simulink model "power_theft_simulink_2"  (R2026a)
settings: Solver=ode23t  StopTime=6  MaxStep=1e-4
libraries: fl_lib x14, nesl_utility x7, ee_lib x1
settings Model: Creator=LAKSHMAN  LastModifiedBy=LAKSHMAN

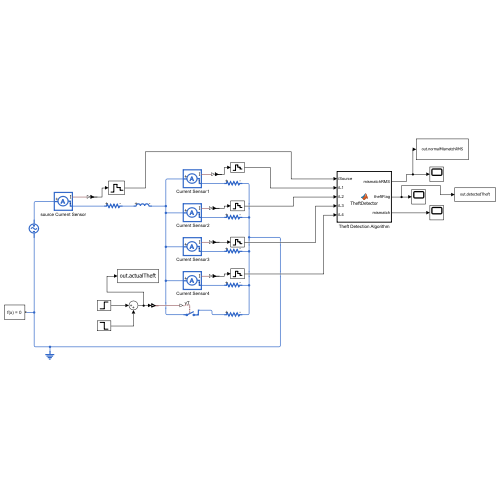
[thumbnail: Simulink's stored preview of the top-level diagram]
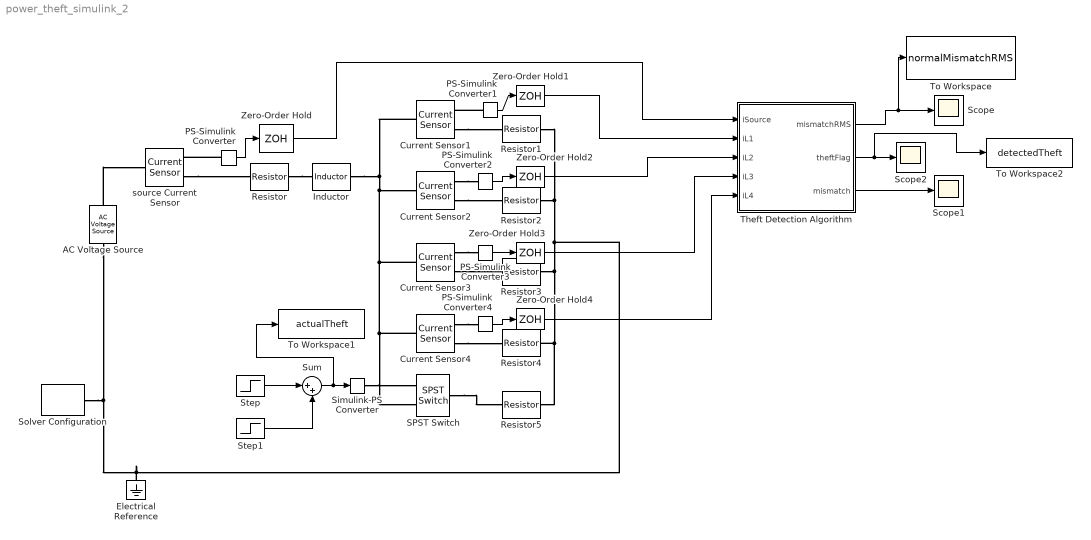
== system power_theft_simulink_2 ==
   Current Sensor{1..4} (4 alike) : fl_lib/Electrical/Electrical Sensors/Current Sensor
  AC Voltage Source : fl_lib/Electrical/Electrical Sources/AC Voltage Source  amp=325.27 V  shift=0 deg  frequency=50 Hz
  Electrical Reference : fl_lib/Electrical/Electrical Elements/Electrical Reference
  Inductor : fl_lib/Electrical/Electrical Elements/Inductor  l=1e-6 H  r=0 Ohm  g=1e-9 1/Ohm  i_specify=off  i_priority=None  i=0 A  i_nominal_specify=off  i_nominal_value=1  i_nominal_unit=A  v_specify=off  v_priority=None  v=0 V  v_nominal_specify=off  v_nominal_value=1  v_nominal_unit=V  i_L_specify=off  i_L_priority=High  i_L=0 A  i_L_nominal_specify=off  i_L_nominal_value=1  i_L_nominal_unit=A
  PS-Simulink Converter{,1..4} (5 alike) : nesl_utility/PS-Simulink Converter  PhysicalDomain=network_engine_domain  SubClassName=ps_output  LeftPortType=input  RightPortType=output  PseudoPeriodic=off  Frequencies=[]  VectorFormat=inherit  Unit=A  AffineConversion=off
  Resistor : fl_lib/Electrical/Electrical Elements/Resistor  R=0.3 Ohm  i_specify=off  i_priority=None  i=0 A  i_nominal_specify=off  i_nominal_value=1  i_nominal_unit=A  v_specify=off  v_priority=None  v=0 V  v_nominal_specify=off  v_nominal_value=1  v_nominal_unit=V
  Resistor1 : fl_lib/Electrical/Electrical Elements/Resistor  R=115 Ohm  i_specify=off  i_priority=None  i=0 A  i_nominal_specify=off  i_nominal_value=1  i_nominal_unit=A  v_specify=off  v_priority=None  v=0 V  v_nominal_specify=off  v_nominal_value=1  v_nominal_unit=V
  Resistor2 : fl_lib/Electrical/Electrical Elements/Resistor  R=76.67 Ohm  i_specify=off  i_priority=None  i=0 A  i_nominal_specify=off  i_nominal_value=1  i_nominal_unit=A  v_specify=off  v_priority=None  v=0 V  v_nominal_specify=off  v_nominal_value=1  v_nominal_unit=V
  Resistor3 : fl_lib/Electrical/Electrical Elements/Resistor  R=57.5 Ohm  i_specify=off  i_priority=None  i=0 A  i_nominal_specify=off  i_nominal_value=1  i_nominal_unit=A  v_specify=off  v_priority=None  v=0 V  v_nominal_specify=off  v_nominal_value=1  v_nominal_unit=V
  Resistor4 : fl_lib/Electrical/Electrical Elements/Resistor  R=153.33 Ohm  i_specify=off  i_priority=None  i=0 A  i_nominal_specify=off  i_nominal_value=1  i_nominal_unit=A  v_specify=off  v_priority=None  v=0 V  v_nominal_specify=off  v_nominal_value=1  v_nominal_unit=V
  Resistor5 : fl_lib/Electrical/Electrical Elements/Resistor  R=115 Ohm  i_specify=off  i_priority=None  i=0 A  i_nominal_specify=off  i_nominal_value=1  i_nominal_unit=A  v_specify=off  v_priority=None  v=0 V  v_nominal_specify=off  v_nominal_value=1  v_nominal_unit=V
  SPST Switch : ee_lib/Switches & Breakers/SPST Switch  R_closed=0.01 Ohm  G_open=1e-6 S  Threshold=0.5 V  Width=0 V  model_dynamics=0  t_on=1e-3 s  t_off=1e-3 s  initial_vT=0 V
  Scope : Scope
      settings: ActiveDisplayYMinimum=-0.16610294723322627  ActiveDisplayYMaximum=2.1764557955338244
  Scope1 : Scope
      settings: ActiveDisplayYMinimum=-0.28618079873529312  ActiveDisplayYMaximum=0.609056055557449
  Scope2 : Scope
      settings: ActiveDisplayYMinimum=-0.044781098945684605  ActiveDisplayYMaximum=1.2677189010543157  DataLoggingVariableName=ScopeData2
  Simulink-PS Converter : nesl_utility/Simulink-PS Converter  PhysicalDomain=network_engine_domain  SubClassName=ps_input  LeftPortType=input  RightPortType=output  PseudoPeriodic=off  Frequencies=[]  NoiseDistribution=none  NoiseParameters=[]  Unit=1  AffineConversion=off  FilteringAndDerivatives=provide  SimscapeFilterOrder=1  InputFilterTimeConstant=0.001  UdotUserProvided=0
  Solver Configuration : nesl_utility/Solver Configuration  PhysicalDomain=network_engine_domain  SubClassName=solver  LeftPortType=input  RightPortType=generic  Tones=[]  Harmonics=[]  SimulateNoise=off  Profile=off  UseLocalSampling=off  EnableSwitchedLinearOptims=on  FrequencyDomain=off  UseCCode=off  RelTol=0.001  AbsTol=0.001  MinStep=1e-09  ToWorkspace=off  RevertToSquareIcSolve=off  NumHomotopyIterations=100  PhasorMode=off  PhasorModeNumHarmonics=1  ConsistencySolver=NEWTON_XTOL_AFTER_FTOL  CanonicalOrdering=CANONICAL  OptimizeIntermediates=OPTIMIZED  IndexReductionMethod=DerivativeReplacement  DoDC=off  ResidualTolerance=1e-09  ConsistencyTolSource=GLOBAL  ConsistencyAbsTol=0.001  ConsistencyRelTol=0.001  ConsistencyTolFactor=0.001  UseLocalSolver=off  LocalSolverChoice=NE_BACKWARD_EULER_ADVANCER  ResolveIndetEquations=on  FunctionEvalNumThread=1  LocalSolverSampleTime=0.001  DoFixedCost=off  MaxNonlinIter=3  MaxModeIter=2  ComputeImpulses=off  ImpulseIterations=2  LinearAlgebra=auto  LinearAlgebraNumThread=0  EquationFormulation=NE_TIME_EF  DelaysMemoryBudget=1024  AutomaticFiltering=on  FilteringTimeConstant=0.001  PartitionStorageMethod=AS_NEEDED  PartitionMemoryBudget=1024  PartitionMethod=ROBUST  MultibodyUseLocalSolver=off  MultibodyLocalSolverChoice=ODE1  MultibodyLocalSolverSampleTime=0.001
  Step : Step  Time=2  SampleTime=0
  Step1 : Step  Time=4.2  FinalValue=-1  SampleTime=0
  Sum : Sum  Inputs=|++
  Theft Detection Algorithm : MATLAB Function  TreatAsAtomicUnit=on
  To Workspace : ToWorkspace  VariableName=normalMismatchRMS  SaveFormat=Timeseries  SampleTime=-1
  To Workspace1 : ToWorkspace  VariableName=actualTheft  SaveFormat=Timeseries  SampleTime=-1
  To Workspace2 : ToWorkspace  VariableName=detectedTheft  SaveFormat=Timeseries  SampleTime=-1
  Zero-Order Hold{,1..4} (5 alike) : ZeroOrderHold  SampleTime=0.0005
  source Current Sensor : fl_lib/Electrical/Electrical Sensors/Current Sensor
  wires:
  Step/1 -> Sum/1
  Step1/1 -> Sum/2
  Sum/1 -> To Workspace1/1, Simulink-PS Converter/1
  PS-Simulink Converter3/1 -> Zero-Order Hold3/1
  PS-Simulink Converter4/1 -> Zero-Order Hold4/1
  PS-Simulink Converter2/1 -> Zero-Order Hold2/1
  PS-Simulink Converter1/1 -> Zero-Order Hold1/1
  PS-Simulink Converter/1 -> Zero-Order Hold/1
  Zero-Order Hold/1 -> Theft Detection Algorithm/1(iSource)
  Zero-Order Hold1/1 -> Theft Detection Algorithm/2(iL1)
  Zero-Order Hold2/1 -> Theft Detection Algorithm/3(iL2)
  Zero-Order Hold3/1 -> Theft Detection Algorithm/4(iL3)
  Zero-Order Hold4/1 -> Theft Detection Algorithm/5(iL4)
  Theft Detection Algorithm/1(mismatchRMS) -> To Workspace/1, Scope/1
  Theft Detection Algorithm/3(mismatch) -> Scope1/1
  Theft Detection Algorithm/2(theftFlag) -> To Workspace2/1, Scope2/1
  connections:
  " Current Sensor1"/RConn2 -- Resistor1/LConn1
  " Current Sensor2"/RConn2 -- Resistor2/LConn1
  " Current Sensor3"/RConn2 -- Resistor3/LConn1
  " Current Sensor4"/RConn2 -- Resistor4/LConn1
  " Current Sensor1"/LConn1 -- Inductor/RConn1 -- " Current Sensor4"/LConn1 -- SPST Switch/LConn2 -- " Current Sensor3"/LConn1 -- " Current Sensor2"/LConn1
  Resistor/RConn1 -- Inductor/LConn1
  source Current Sensor/RConn2 -- Resistor/LConn1
  AC Voltage Source/LConn1 -- source Current Sensor/LConn1
  Resistor1/RConn1 -- Resistor2/RConn1 -- Resistor5/RConn1 -- Resistor4/RConn1 -- Resistor3/RConn1 -- Solver Configuration/RConn1 -- AC Voltage Source/RConn1 -- Electrical Reference/LConn1
  Simulink-PS Converter/RConn1 -- SPST Switch/LConn1
  PS-Simulink Converter/LConn1 -- source Current Sensor/RConn1
  PS-Simulink Converter1/LConn1 -- " Current Sensor1"/RConn1
  " Current Sensor2"/RConn1 -- PS-Simulink Converter2/LConn1
  " Current Sensor3"/RConn1 -- PS-Simulink Converter3/LConn1
  " Current Sensor4"/RConn1 -- PS-Simulink Converter4/LConn1
  SPST Switch/RConn1 -- Resistor5/LConn1

== matlab function power_theft_simulink_2/Theft Detection Algorithm ==
  data: iSource input; mismatchRMS output; iL1 input; iL2 input; iL3 input; iL4 input; theftFlag output; mismatch output
function [mismatchRMS, theftFlag, mismatch] = ...
    TheftDetector(iSource, iL1, iL2, iL3, iL4)
%#codegen

N = 200;              % 100 ms at 2000 Hz
thresholdA = 0.20;    % Initial threshold in amperes

persistent buffer idx sumSq count

if isempty(buffer)
    buffer = zeros(N,1);
    idx = 1;
    sumSq = 0.0;
    count = 0;
end

% Current not accounted for by the four registered consumers
mismatch = iSource - (iL1 + iL2 + iL3 + iL4);

% Maintain a rolling sum of squared mismatch samples
newSq = mismatch * mismatch;
oldSq = buffer(idx);

buffer(idx) = newSq;
sumSq = sumSq - oldSq + newSq;

idx = idx + 1;
if idx > N
    idx = 1;
end

if count < N
    count = count + 1;
end

% RMS mismatch over the available trailing samples
mismatchRMS = sqrt(max(sumSq / count, 0));

% Alarm flag: 1 = suspected theft, 0 = no alarm
theftFlag = double(mismatchRMS > thresholdA);
end
